simulink model "reference_feedback"  (R2026b)
settings: Solver=FixedStepDiscrete  StartTime=0  StopTime=0.4  FixedStep=0.1
settings Model: Creator=Fasih  LastModifiedBy=Fasih

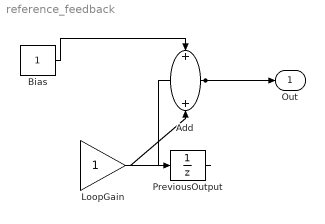
== system reference_feedback ==
  Add : Sum
  Bias : Constant
  LoopGain : Gain
  PreviousOutput : UnitDelay  SampleTime=0.1
  Out : Outport
  wires:
  Bias/1 -> Add/1
  PreviousOutput/1 -> LoopGain/1
  LoopGain/1 -> Add/2
  Add/1 -> Out/1, PreviousOutput/1
